simulink model "SMC_simulation"  (R2025a)
settings: Solver=ode4  StartTime=0.0  StopTime=200  FixedStep=1e-3  MaxStep=1e-2  MinStep=1e-6  RelTol=1e-6
undefined symbols (not defined in the file or in its folder): p
settings Model: Creator=Giammo  LastModifiedBy=Giammo
settings SolverCC: InitialStep=1e-6  ZeroCrossControl=EnableAll  ZeroCrossAlgorithm=Adaptive  SolverResetMethod=Robust

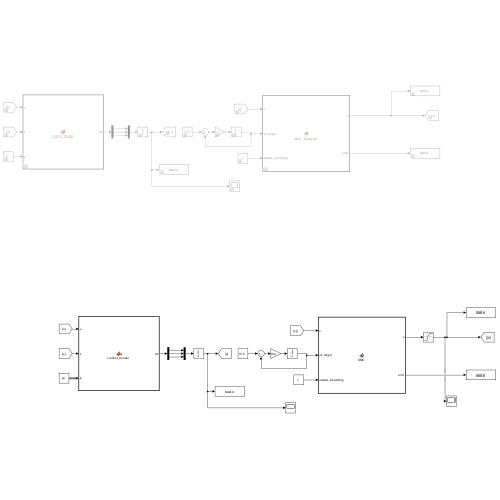
[thumbnail: Simulink's stored preview of the top-level diagram]
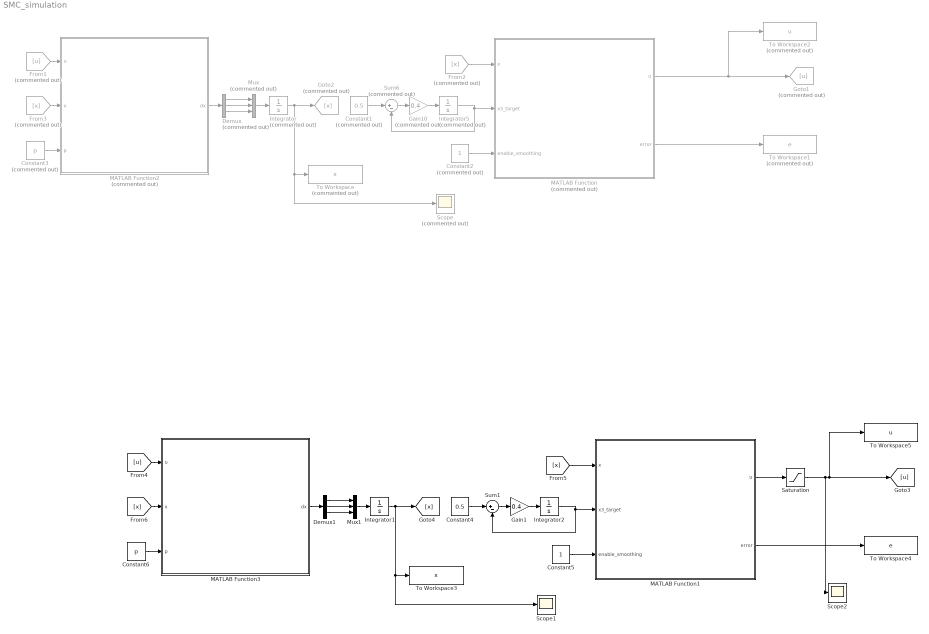
== system SMC_simulation ==
  Constant1 : Constant  Commented=on  Value=0.5
  Constant2 : Constant  Commented=on
  Constant3 : Constant  Commented=on  Value=p  OutDataTypeStr=Bus: slBus1
  Constant4 : Constant  Value=0.5
  Constant5 : Constant
  Constant6 : Constant  Value=p  OutDataTypeStr=Bus: slBus1
  Demux : Demux  Commented=on  Outputs=3
  Demux1 : Demux  Outputs=3
  From1 : From  Commented=on  GotoTag=u
  From2 : From  Commented=on  GotoTag=x
  From3 : From  Commented=on  GotoTag=x
  Gain1 : Gain  Gain=0.4
  Gain10 : Gain  Commented=on  Gain=0.4
  Goto1 : Goto  Commented=on  GotoTag=u
  Goto2 : Goto  Commented=on  GotoTag=x
  Integrator : Integrator  Commented=on  InitialCondition=[0.9;0.1;0.1]
  Integrator1 : Integrator  InitialCondition=[0.1;0.1;0.1]
  Integrator2 : Integrator  InitialCondition=0.4
  Integrator5 : Integrator  Commented=on  InitialCondition=0.5
  MATLAB Function : MATLAB Function  Commented=on  TreatAsAtomicUnit=on
  MATLAB Function1 : MATLAB Function  TreatAsAtomicUnit=on
  MATLAB Function2 : MATLAB Function  Commented=on  TreatAsAtomicUnit=on
  MATLAB Function3 : MATLAB Function  TreatAsAtomicUnit=on
  Mux : Mux  Commented=on  Inputs=3
  Mux1 : Mux  Inputs=3
  Saturation : Saturate  UpperLimit=1  LowerLimit=0
  Scope : Scope  Commented=on
      settings: ActiveDisplayYMinimum=-0.12499999999998841  ActiveDisplayYMaximum=1.1249999999998959
  Scope1 : Scope
      settings: ActiveDisplayYMinimum=-0.12499999999998841  ActiveDisplayYMaximum=1.1249999999998959
  Scope2 : Scope
      settings: ActiveDisplayYMinimum=-0.12499999999999997  ActiveDisplayYMaximum=1.125  DataLoggingVariableName=ScopeData2
  Sum1 : Sum  Inputs=|+-
  Sum6 : Sum  Commented=on  Inputs=|+-
  To Workspace : ToWorkspace  Commented=on  VariableName=x  SaveFormat=Timeseries  SampleTime=-1
  To Workspace1 : ToWorkspace  Commented=on  VariableName=e  SaveFormat=Timeseries  SampleTime=-1
  To Workspace2 : ToWorkspace  Commented=on  VariableName=u  SaveFormat=Timeseries  SampleTime=-1
  To Workspace3 : ToWorkspace  VariableName=x  SaveFormat=Timeseries  SampleTime=-1
  To Workspace4 : ToWorkspace  VariableName=e  SaveFormat=Timeseries  SampleTime=-1
  To Workspace5 : ToWorkspace  VariableName=u  SaveFormat=Timeseries  SampleTime=-1
  wires:
  Constant3/1 -> MATLAB Function2/3(p)
  Sum6/1 -> Gain10/1
  Constant1/1 -> Sum6/1
  Integrator5/1 -> Sum6/2, MATLAB Function/2(x3_target)
  Gain10/1 -> Integrator5/1
  Constant2/1 -> MATLAB Function/3(enable_smoothing)
  From2/1 -> MATLAB Function/1(x)
  From3/1 -> MATLAB Function2/2(x)
  Integrator/1 -> Goto2/1, Scope/1, To Workspace/1
  MATLAB Function2/1(dx) -> Demux/1
  Demux/2 -> Mux/2
  Mux/1 -> Integrator/1
  MATLAB Function/2(error) -> To Workspace1/1
  Demux/3 -> Mux/3
  MATLAB Function/1(u) -> To Workspace2/1, Goto1/1
  Demux/1 -> Mux/1
  From1/1 -> MATLAB Function2/1(u)
  [u] -> MATLAB Function3/1(u)
  Demux1/1 -> Mux1/1
  Constant4/1 -> Sum1/1
  MATLAB Function1/1(u) -> Saturation/1
  [x] -> MATLAB Function1/1(x)
  Sum1/1 -> Gain1/1
  Constant5/1 -> MATLAB Function1/3(enable_smoothing)
  [x] -> MATLAB Function3/2(x)
  Demux1/2 -> Mux1/2
  Integrator2/1 -> Sum1/2, MATLAB Function1/2(x3_target)
  Integrator1/1 -> [x], Scope1/1, To Workspace3/1
  Constant6/1 -> MATLAB Function3/3(p)
  Mux1/1 -> Integrator1/1
  MATLAB Function3/1(dx) -> Demux1/1
  Gain1/1 -> Integrator2/1
  MATLAB Function1/2(error) -> To Workspace4/1
  Saturation/1 -> Scope2/1, To Workspace5/1, [u]
  Demux1/3 -> Mux1/3

== matlab function SMC_simulation/MATLAB Function1 ==
  data: x input; u output; x3_target input; enable_smoothing input; error output
function [u,error] = SMC(x, x3_target, enable_smoothing)
    % Regulate the resting-cell population around x3_target.
    R3 = 4.5; D3 = 0.5; A31 = 0.2; k3 = 1.0;
    
    x1 = x(1);
    x3 = x(3); 
    
    lambda = 2.0; 
    % Define the sliding variable from the resting-cell tracking error.
    sigma = lambda * (x3 - x3_target);
    error = x3 - x3_target;

    f3 = (R3 * x1 * x3) / (x1 + k3) - A31 * x1 * x3 - D3 * x3;
    K = 50.0; 
    u_eq = -f3; 
    
    % Select sign switching or a smooth tanh approximation.
    if enable_smoothing == 0
        u_sw = -(K / lambda) * sign(sigma);
    else
        phi = 1; 
        u_sw = -(K / lambda) * tanh(sigma / phi);
    end
    
    u_ideal = u_eq + u_sw;
    u = u_ideal;
end

== matlab function SMC_simulation/MATLAB Function ==
  data: x input; u output; x3_target input; enable_smoothing input; error output
function [u,error] = SMC_Dualmod(x, x3_target, enable_smoothing)
    % Sliding mode control with separate stimulation and inhibition limits.
   
    R3  = 4.5; D3  = 0.5; A31 = 0.2; k3  = 1.0;
    
    x1 = x(1); 
    x3 = x(3); 
    
    
    u_max_stim = 1.0;   
    u_max_inh  = -1.0;  
    
   
    lambda = 1.0; 
    sigma = lambda * (x3 - x3_target);
    error = x3 - x3_target;
    f3_drift = (R3 * x1 * x3) / (x1 + k3) - A31 * x1 * x3 - D3 * x3;
    Lf_sigma = lambda * f3_drift;
    Lg_sigma = lambda; 
    % Equivalent control cancels the nominal drift on the sliding surface.
    u_eq = -Lf_sigma / Lg_sigma;
    K = 1;
    % Select sign switching or a smooth tanh approximation.
    if enable_smoothing == 0
        u_sw = -(K / Lg_sigma) * sign(sigma);
    else
        phi = 1; 
        u_sw = -(K / Lg_sigma) * tanh(sigma / phi);
    end 
    u_ideal = u_eq + u_sw;
        u_stim = 0;
    u_inhib = 0;
    % Saturate the control channel selected by the command sign.
    if u_ideal >= 0
        u_stim_raw = u_ideal;
        u_stim = min(u_stim_raw, u_max_stim); 
        u_inhib = 0;
    else
        u_inhib_raw = u_ideal;
        u_inhib = max(u_inhib_raw, u_max_inh);     
        u_stim = 0;
    end
    u = u_stim + u_inhib;

end

== matlab function SMC_simulation/MATLAB Function2 ==
  data: u input; dx output; x input; p input
function dx = cancer_model(u, x, p)
    % Continuous-time dynamics: states are tumor, hunting cells and resting cells; u acts on x3.

    x1 = x(1);
    x2 = x(2);
    x3 = x(3);
    A12 = p.A12;
    A13 = p.A13;
    R2  = p.R2;
    A21 = p.A21;
    R3  = p.R3;
    k3  = p.k3;
    A31 = p.A31;
    D3  = p.D3;
    dx = zeros(3,1);
    dx(1) = x1*(1 - x1) - A12*x1*x2 - A13*x1*x3;
    dx(2) = R2*x2*(1 - x2) - A21*x1*x2;
    recruitment = (R3 * x1 * x3) / (x1 + k3);
    dx(3) = recruitment - A31*x1*x3 - D3*x3 + u;

end

== matlab function SMC_simulation/MATLAB Function3 ==
  data: u input; dx output; x input; p input
function dx = cancer_model(u, x, p)
    % Continuous-time dynamics: states are tumor, hunting cells and resting cells; u acts on x3.

    x1 = x(1);
    x2 = x(2);
    x3 = x(3);
    A12 = p.A12;
    A13 = p.A13;
    R2  = p.R2;
    A21 = p.A21;
    R3  = p.R3;
    k3  = p.k3;
    A31 = p.A31;
    D3  = p.D3;
    dx = zeros(3,1);
    dx(1) = x1*(1 - x1) - A12*x1*x2 - A13*x1*x3;
    dx(2) = R2*x2*(1 - x2) - A21*x1*x2;
    recruitment = (R3 * x1 * x3) / (x1 + k3);
    dx(3) = recruitment - A31*x1*x3 - D3*x3 + u;

end
